simulink model "huizhenglijujisuan_zuixin"  (R2024b)
settings: Solver=FixedStepAuto  StartTime=0.0  StopTime=10  FixedStep=1e-4  MaxStep=1e-2  RelTol=1e-3
model workspace (MAT data in the model file):
  angle : Simulink.Parameter (value not decoded)
libraries: simulink x4, spsPermanentMagnetSynchronousMachineLib x2, slpidlib x2, powerlib_extras x2, Solver_SF x1, spsDCVoltageSourceLib x1, spsUniversalBridgeLib x1, spspowerguiLib x1
(part 2 of 2)

== matlab function huizhenglijujisuan_zuixin/PAC1/rr ==
  data: Fz input; alpha input; Fy0 output; Mz output
function [Fy0,Mz] = tire(Fz,alpha)
if Fz>0
%Fz 轮胎垂向载荷 N
%camber 外倾角 rad？？？
%lamda 纵向滑移率
%alpha 车辆侧偏角 rad
alpha=tan(alpha);
camber=0;
Fz0=8000; %名义垂向载荷N
dfz=(Fz-Fz0)/Fz0;
% %% Pure_Fx
% %轮胎参数——纵向力
% pcx1=1.65;
% pdx1=1.3; pdx2=-0.15; pdx3=0;
% pex1=0; pex2=0;pex3=0; pex4=0;
% pkx1=20; pkx2=0; pkx3=0;
% pvx1=0; pvx2=0;
% phx1=0; phx2=0;
% %pure_Fx 魔术公式
% Cx=pcx1;
% Shx=phx1+phx2*dfz;
% lamda_x=lamda+Shx;
% Dx=(pdx1+pdx2*dfz)*(1-pdx3*camber*camber)*Fz;
% Ex=(pex1+pex2*dfz+pex3*dfz*dfz)*(1-pex4*sign(lamda_x));
% Kx=Fz*(pkx1+pkx2*dfz)*exp(pkx3*dfz);
% Bx=Kx/(Cx*Dx);
% Svx=Fz*(pvx1+pvx2*dfz);
% Fx0=Dx*sin(Cx*atan(Bx*lamda_x-Ex*(Bx*lamda_x-atan(Bx*lamda_x))))+Svx;
% %% 联合工况纵向力Fx
% %轮胎参数——纵向力
% rbx1=20;rbx2=15;
% rcx1=1;
% rex1=0;rex2=0;
% rhx1=0;
% %纵向力加权函数
% Bxa=rbx1*cos(atan(rbx2*lamda));
% Cxa=rcx1;
% Exa=rex1+rex2*dfz;
% Shxa=rhx1;
% alpha_s=alpha+Shxa;
% Gxa=cos(Cxa*atan(Bxa*alpha_s-Exa*(Bxa*alpha_s-atan(Bxa*alpha_s))))/cos(Cxa*atan(Bxa*Shxa-Exa*(Bxa*Shxa-atan(Bxa*Shxa))));
% Fx=Fx0*Gxa;



%% Pure_Fy
%轮胎参数——侧向力
pcy1=1.529245171;
pdy1=1.038581713; pdy2=-0.179464279; pdy3=-0.683745879;
pey1=-0.39012519; pey2=-0.611160145;pey3=-0.040677215; pey4=-14.95422065;
pky1=-26.056726760; pky2=2.106504624; pky3=0.499984439;
pvy1=0; pvy2=0;pvy3=0;pvy4=0;
phy1=0; phy2=0;phy3=0;
%pure_Fy 魔术公式
Cy=pcy1;
Shy=phy1+phy2*dfz+phy3*camber;
alpha_y=alpha+Shy;
uy=(pdy1+pdy2*dfz)*(1-pdy3*camber*camber);
Dy=uy*Fz;
Ey=(pey1+pey2*dfz)*(1-(pey3+pey4*camber)*sign(alpha_y));
Ky=pky1*Fz0*sin(2*atan(Fz/(pky2*Fz0)))*(1-pky3*abs(camber));
By=Ky/(Cy*Dy);
Svy=Fz*(pvy1+pvy2*dfz+(pvy3+pvy4*dfz)*camber);
Fy0=Dy*sin(Cy*atan(By*alpha_y-Ey*(By*alpha_y-atan(By*alpha_y))))+Svy;
% %% 联合工况侧向力Fy
% %轮胎参数——侧向力
% rby1=10;rby2=10;rby3=-0.027856;
% rcy1=1;
% rey1=0;rey2=0;
% rhy1=0;rhy2=0;
% rvy1=0;rvy2=0;rvy3=0;rvy4=20;rvy5=2;rvy6=10;
% %侧向力加权函数
% Bya=rby1*cos(atan(rby2*(alpha-rby3)));
% Cya=rcy1;
% Eya=rey1+rey2*dfz;
% Shya=rhy1+rhy2*dfz;
% lamda_s=lamda+Shya;
% Gya=cos(Cya*atan(Bya*lamda_s-Eya*(Bya*lamda_s-atan(Bya*lamda_s))))/cos(Cya*atan(Bya*Shya-Eya*(Bya*Shya-atan(Bya*Shya))));
% %轮胎参数——侧向力
% Svyr=uy*Fz*(rvy1+rvy2*dfz+rvy3*camber)*cos(atan(rvy4*alpha))*sin(rvy5*atan(rvy6*lamda));
% Fy=Fy0*Gya+Svyr;

%% Pure_Mz
%轮胎参数——回正力矩
R0=0.357; %轮胎空载半径/m
qbz1=8.37;qbz2=-2.92;qbz3=0.48;qbz4=-0.45;qbz5=-0.44;
qcz1=1.19;
qdz1=0.11;qdz2=-0.003;qdz3=-0.56;qdz4=8.4;
qez1=-2.9;qez2=-0.55;qez3=0;qez4=-0.13;qez5=-3.68;
%pure_Mz0 魔术公式
Ct=qcz1;
alpha_t=alpha;
Bt=(qbz1+qbz2*dfz+qbz3*dfz^2)*(1+qbz4*camber+qbz5*abs(camber));
Dt=Fz*(qdz1+qdz2*dfz)*(1+qdz3*camber+qdz4*camber^2)*R0/Fz0;
Et=(qez1+qez2*dfz+qez3*dfz^2)*(1+(qez4+qez5*camber)*((2/pi)*atan(Bt*Ct*alpha_t)));
t=Dt*cos(Ct*atan(Bt*alpha_t-Et*(Bt*alpha_t-atan(Bt*alpha_t))))*cos(alpha); %轮胎拖距
% 轮胎参数——回正力矩
qbz9=3.44;qbz10=0;
qdz6=0.003;qdz7=0.005;qdz8=-0.12;qdz9=0.12;
Br=(qbz9+qbz10*By*Cy);
Cr=1;
Dr=Fz*(qdz6+qdz7*dfz+(qdz8+qdz9*dfz)*camber)*R0;
alpha_r=alpha;
Mzr=Dr*cos(Cr*atan(Br*alpha_r))*cos(alpha); %残余力矩
Mz=-t*Fy0+Mzr;
else
    Fx0=0;
    Fy0=0;
    Fx=0;
    Fy=0;
    Mz=0;
end

== matlab function huizhenglijujisuan_zuixin/MATLAB Function ==
  data: Tsw input; Tz output; v input
function Tz = fcn(Tsw,v)
Tz=0;
if v>5&&v<=50
    a=1.35;
elseif v<=5
    a=2.2;
else
    a=1.35;
end

kv=exp(-(v/160)^2)*40;
% gv=((Tsw-1)/(7-1))^a;
if Tsw<=1&&Tsw>-1
        Tz=0;
end

if Tsw>1&&Tsw<7
        Tz=kv*((Tsw-1)/(7-1))^a;
end

if Tsw>=7
        Tz=kv;
end

if Tsw>-7&&Tsw<-1
        Tz=-kv*((-Tsw-1)/(7-1))^a;
end

if Tsw<=-7
        Tz=-kv;
end
end

== matlab function huizhenglijujisuan_zuixin/PAC1/fl ==
  data: Fz input; alpha input; Fy0 output; Mz output; Mzr output; t output; M1 output; Mznew output
function [Fy0,Mz,Mzr,t,M1,Mznew] = tire(Fz,alpha)
t=0;
Mzr=0;
if Fz>0
%Fz 轮胎垂向载荷 N
%camber 外倾角 rad？？？
%lamda 纵向滑移率
%alpha 车辆侧偏角 rad
alpha=tan(alpha);
camber=0;
Fz0=8000; %名义垂向载荷N
dfz=(Fz-Fz0)/Fz0;
% %% Pure_Fx
% %轮胎参数——纵向力
% pcx1=1.65;
% pdx1=1.3; pdx2=-0.15; pdx3=0;
% pex1=0; pex2=0;pex3=0; pex4=0;
% pkx1=20; pkx2=0; pkx3=0;
% pvx1=0; pvx2=0;
% phx1=0; phx2=0;
% %pure_Fx 魔术公式
% Cx=pcx1;
% Shx=phx1+phx2*dfz;
% lamda_x=lamda+Shx;
% Dx=(pdx1+pdx2*dfz)*(1-pdx3*camber*camber)*Fz;
% Ex=(pex1+pex2*dfz+pex3*dfz*dfz)*(1-pex4*sign(lamda_x));
% Kx=Fz*(pkx1+pkx2*dfz)*exp(pkx3*dfz);
% Bx=Kx/(Cx*Dx);
% Svx=Fz*(pvx1+pvx2*dfz);
% Fx0=Dx*sin(Cx*atan(Bx*lamda_x-Ex*(Bx*lamda_x-atan(Bx*lamda_x))))+Svx;
% %% 联合工况纵向力Fx
% %轮胎参数——纵向力
% rbx1=20;rbx2=15;
% rcx1=1;
% rex1=0;rex2=0;
% rhx1=0;
% %纵向力加权函数
% Bxa=rbx1*cos(atan(rbx2*lamda));
% Cxa=rcx1;
% Exa=rex1+rex2*dfz;
% Shxa=rhx1;
% alpha_s=alpha+Shxa;
% Gxa=cos(Cxa*atan(Bxa*alpha_s-Exa*(Bxa*alpha_s-atan(Bxa*alpha_s))))/cos(Cxa*atan(Bxa*Shxa-Exa*(Bxa*Shxa-atan(Bxa*Shxa))));
% Fx=Fx0*Gxa;



%% Pure_Fy
%轮胎参数——侧向力
pcy1=1.529245171;
pdy1=1.038581713; pdy2=-0.179464279; pdy3=-0.683745879;
pey1=-0.39012519; pey2=-0.611160145;pey3=-0.040677215; pey4=-14.95422065;
pky1=-26.056726760; pky2=2.106504624; pky3=0.499984439;
pvy1=0; pvy2=0;pvy3=0;pvy4=0;
phy1=0; phy2=0;phy3=0;
%pure_Fy 魔术公式
Cy=pcy1;
Shy=phy1+phy2*dfz+phy3*camber;
alpha_y=alpha+Shy;
uy=(pdy1+pdy2*dfz)*(1-pdy3*camber*camber);
Dy=uy*Fz;
Ey=(pey1+pey2*dfz)*(1-(pey3+pey4*camber)*sign(alpha_y));
Ky=pky1*Fz0*sin(2*atan(Fz/(pky2*Fz0)))*(1-pky3*abs(camber));
By=Ky/(Cy*Dy);
Svy=Fz*(pvy1+pvy2*dfz+(pvy3+pvy4*dfz)*camber);
Fy0=Dy*sin(Cy*atan(By*alpha_y-Ey*(By*alpha_y-atan(By*alpha_y))))+Svy;
% %% 联合工况侧向力Fy
% %轮胎参数——侧向力
% rby1=10;rby2=10;rby3=-0.027856;
% rcy1=1;
% rey1=0;rey2=0;
% rhy1=0;rhy2=0;
% rvy1=0;rvy2=0;rvy3=0;rvy4=20;rvy5=2;rvy6=10;
% %侧向力加权函数
% Bya=rby1*cos(atan(rby2*(alpha-rby3)));
% Cya=rcy1;
% Eya=rey1+rey2*dfz;
% Shya=rhy1+rhy2*dfz;
% lamda_s=lamda+Shya;
% Gya=cos(Cya*atan(Bya*lamda_s-Eya*(Bya*lamda_s-atan(Bya*lamda_s))))/cos(Cya*atan(Bya*Shya-Eya*(Bya*Shya-atan(Bya*Shya))));
% %轮胎参数——侧向力
% Svyr=uy*Fz*(rvy1+rvy2*dfz+rvy3*camber)*cos(atan(rvy4*alpha))*sin(rvy5*atan(rvy6*lamda));
% Fy=Fy0*Gya+Svyr;

%% Pure_Mz
%轮胎参数——回正力矩
R0=0.357; %轮胎空载半径/m
qbz1=8.37;qbz2=-2.92;qbz3=0.48;qbz4=-0.45;qbz5=-0.44;
qcz1=1.19;
qdz1=0.11;qdz2=-0.003;qdz3=-0.56;qdz4=8.4;
qez1=-2.9;qez2=-0.55;qez3=0;qez4=-0.13;qez5=-3.68;
%pure_Mz0 魔术公式
Ct=qcz1;
alpha_t=alpha;
Bt=(qbz1+qbz2*dfz+qbz3*dfz^2)*(1+qbz4*camber+qbz5*abs(camber));
Dt=Fz*(qdz1+qdz2*dfz)*(1+qdz3*camber+qdz4*camber^2)*R0/Fz0;
Et=(qez1+qez2*dfz+qez3*dfz^2)*(1+(qez4+qez5*camber)*((2/pi)*atan(Bt*Ct*alpha_t)));
t=Dt*cos(Ct*atan(Bt*alpha_t-Et*(Bt*alpha_t-atan(Bt*alpha_t))))*cos(alpha); %轮胎拖距
% 轮胎参数——回正力矩
qbz9=3.44;qbz10=0;
qdz6=0.003;qdz7=0.005;qdz8=-0.12;qdz9=0.12;
Br=(qbz9+qbz10*By*Cy);
Cr=1;
Dr=Fz*(qdz6+qdz7*dfz+(qdz8+qdz9*dfz)*camber)*R0;
alpha_r=alpha;
Mzr=Dr*cos(Cr*atan(Br*alpha_r))*cos(alpha); %残余力矩
M1=-R0*tan(5/180*pi)*Fy0;
Mz=-t*Fy0;
Mznew=Mz+M1;
else
    Fx0=0;
    Fy0=0;
    Fx=0;
    Fy=0;
    Mz=0;
    M1=0;
    Mznew=0;
end

== matlab function huizhenglijujisuan_zuixin/MATLAB Function1 ==
  data: v input; Tfric output; dsw input
function Tfric = fcn(v,dsw)
if v<=40
    Tv=0.25;
else
    Tv=0.35;
end
dsw=dsw*pi/180;
kv=100;
Tfric =Tv*tanh(kv*dsw)+0.0005*dsw;

== matlab function huizhenglijujisuan_zuixin/MATLAB Function2 ==
  data: v input; Tzuni output; dsw input
function Tzuni = fcn(v,dsw)
v0=20;
sig=((1+sign(v-v0))/2);
k=0.002;
dsw=dsw*pi/180;
kv=k*(v-v0)/3.6*dsw;
Tzuni=sig*(kv-0.005);

== matlab function huizhenglijujisuan_zuixin/MATLAB Function3 ==
  data: dtsw input; Tguanxing output
function Tguanxing = fcn(dtsw)
J=-0.0008;
Tguanxing=dtsw*J;

== matlab function huizhenglijujisuan_zuixin/MATLAB Function5 ==
  data: sw input; Tlim output
function Tlim = fcn(sw)
k=1;
if abs(sw)>400
    Tlim=k*sign(sw)*(abs(sw)-400)^2;
else
    Tlim=0;
end
